simulink model "apf_system_H2"  (R2025a)
settings: Solver=FixedStepDiscrete  StartTime=0.0  StopTime=T_end  FixedStep=Tps  RelTol=1e-3
PostLoadFcn:
  | addpath(fileparts(get_param('apf_system_H2','FileName'))); if ~exist('P','var'), run(fullfile(fileparts(get_param('apf_system_H2','FileName')),'apf_params.m')); end; if ~exist('S','var'), S = sensor_params_H2; end
InitFcn:
  | addpath(fileparts(get_param('apf_system_H2','FileName'))); if ~exist('P','var'), run(fullfile(fileparts(get_param('apf_system_H2','FileName')),'apf_params.m')); end; if ~exist('S','var'), S = sensor_params_H2; end
values from neighbouring files (symbols this model uses):
  Cdc = 1000e-6    (= 0.001)    [apf_params.m]
  dtc = Td / (Ts / 2) / 2    [apf_params.m]    (also in vps_vectors_H3.m = 0.02)
  f = 50    [apf_params.m]    (also in frontend_sizing_H1.m = fieldnames(opt); sensor_adc_study_H1.m = fullfile(outdir, ['seed777_' s{1} '.csv']); sensor_adc_study_H2.m = fullfile(outdir, [scen{k, 1} '.mat']))
  Lac_load = 0.5e-3    (= 0.0005)    [apf_params.m]
  Ldc_load = 20e-3    (= 0.02)    [apf_params.m]
  Lf = 3e-3    (= 0.003)    [apf_params.m]
  Lgrid = 10e-6    (= 1e-05)    [apf_params.m]
  R_load1 = 33    [apf_params.m]
  R_step = R_load1 * R_load2 / (R_load1 - R_load2)    (= 66)    [apf_params.m]
  Rac_load = 0.01    [apf_params.m]
  Rf = 0.1    [apf_params.m]
  Rgrid = 1e-3    (= 0.001)    [apf_params.m]
  Rleak = 20e3    (= 20000)    [apf_params.m]
  S = struct('tau', [o.tauV o.tauV o.tauI o.tauI o.tauI o.tauI o.tauDC],      'delay', o.delay, 'skew', o.skew, 'conv', o.conv, 'noise', o.noise,      'seed', o.seed, 'adc', logical(o.adc))    [sensor_params_H2.m]    (also in thd_table_H3.m = round(2^15 * sin(2 * pi * m / 200)); vps_rtl_check_H3.m = load(fullfile(outdir, 'vps_runs.mat')))
  T_log = 10e-6    (= 1e-05)    [apf_params.m]
  t_run = 0.01    [apf_params.m]
  t_step = 0.7    [apf_params.m]
  Tps = 0.5e-6    (= 5e-07)    [apf_params.m]    (also in sensor_params_H2.m)
  Ts = P.Ts    [apf_params.m]    (also in sensor_params_H2.m = 0.0001)
  Vll_rms = Vm * sqrt(3) / sqrt(2)    [apf_params.m]
libraries: spsSeriesRLCBranchLib x5, spsThreePhaseVIMeasurementLib x3, spsUniversalBridgeLib x2, spsThreePhaseSeriesRLCBranchLib x2, spsThreePhaseBreakerLib x1, simulink x1, spsThreePhaseSourceLib x1, spsBreakerLib x1, spsVoltageMeasurementLib x1, spspowerguiLib x1
settings Model: Creator=HeKe  LastModifiedBy=HeKe

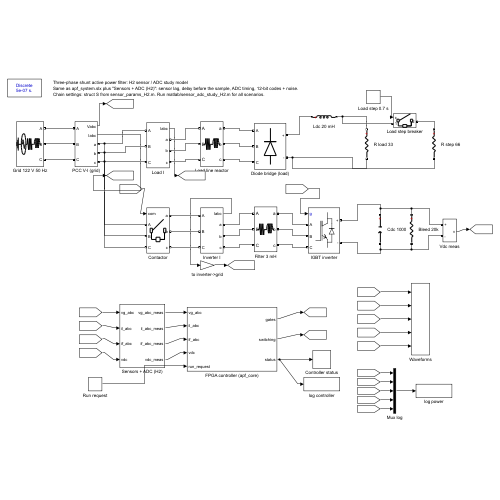
[thumbnail: Simulink's stored preview of the top-level diagram]
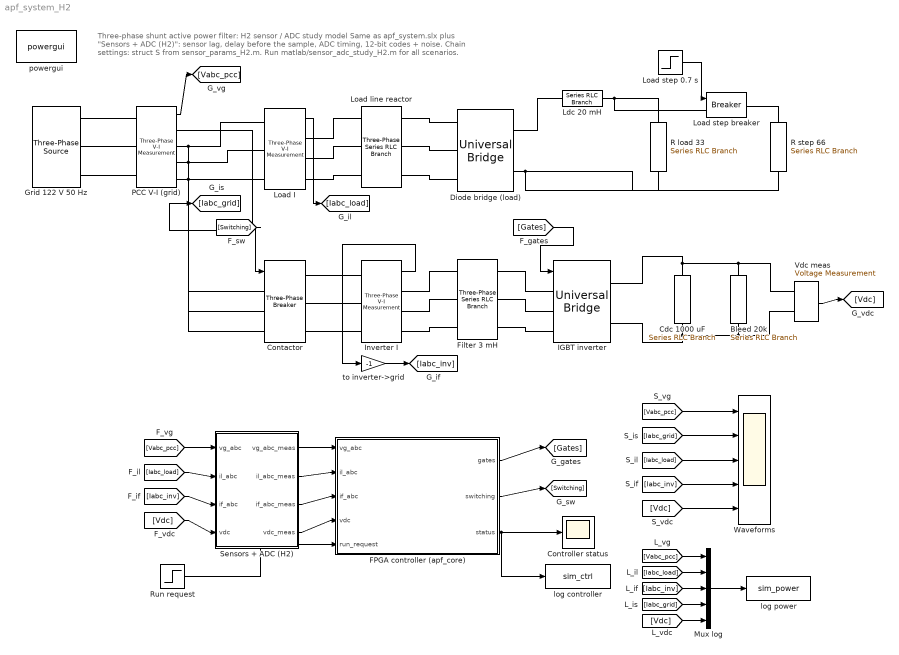
== system apf_system_H2 ==
  note: Three-phase shunt active power filter: H2 sensor / ADC study model
      | Same as apf_system.slx plus "Sensors + ADC (H2)": sensor lag, delay before the sample, ADC timing, 12-bit codes + noise.
      | Chain settings: struct S from sensor_params_H2.m. Run matlab/sensor_adc_study_H2.m for all scenarios.
  Bleed 20k : spsSeriesRLCBranchLib/Series RLC Branch  LConnTagsString=__new0  RConnTagsString=__new0  BranchType=R  Resistance=Rleak  Inductance=1e-3  SetiL0=off  InitialCurrent=0  Capacitance=1e-6  Setx0=off  InitialVoltage=0  Measurements=None
  Cdc 1000 uF : spsSeriesRLCBranchLib/Series RLC Branch  LConnTagsString=__new0  RConnTagsString=__new0  BranchType=C  Resistance=1  Inductance=1e-3  SetiL0=off  InitialCurrent=0  Capacitance=Cdc  Setx0=on  InitialVoltage=Vdc0  Measurements=None
  Contactor : spsThreePhaseBreakerLib/Three-Phase Breaker  InitialState=open  SwitchA=on  SwitchB=on  SwitchC=on  SwitchTimes="[1/60  5/60]"  External=on  BreakerResistance=1e-3  SnubberResistance=1e6  SnubberCapacitance=inf  Measurements=None
  Controller status : Scope
  Diode bridge (load) : spsUniversalBridgeLib/Universal Bridge  Arms=3  SnubberResistance=1e5  SnubberCapacitance=inf  Device=Diodes  Ron=Ron_sw  Lon=0  ForwardVoltages="[  0  0  ]"  ForwardVoltage=0  GTOparameters=[ 10e-6 , 20e-6 ]  IGBTparameters=[ 1e-6 , 2e-6 ]  Measurements=None  Measurements_2=None  converterType=Rectifier
  FPGA controller (apf_core) : Subsystem
  Filter 3 mH : spsThreePhaseSeriesRLCBranchLib/Three-Phase Series RLC Branch  LConnTagsString=A|B|C  RConnTagsString=A|B|C  BranchType=RL  Resistance=Rf  Inductance=Lf  Capacitance=1e-6  Measurements=None
  Grid 122 V 50 Hz : spsThreePhaseSourceLib/Three-Phase Source  InternalConnection=Yg  VoltagePhases=off  Voltage=Vll_rms  PhaseAngle=90  Voltage_phases=[25e3 25e3 25e3]/sqrt(3)  PhaseAngles_phases=[0 -120 +120]  Frequency=f  NonIdealSource=on  SpecifyImpedance=off  Resistance=Rgrid  Inductance=Lgrid  ShortCircuitLevel=100e6  BaseVoltage=25e3  XRratio=7  BusType=swing  Pref=10e3  Qref=0  Prefabc=[10e3, 10e3, 10e3]  Qrefabc=[0, 0, 0]  Qmin=-inf  Qmax=inf
  IGBT inverter : spsUniversalBridgeLib/Universal Bridge  Arms=3  SnubberResistance=1e5  SnubberCapacitance=inf  Device=IGBT / Diodes  Ron=Ron_sw  Lon=0  ForwardVoltages=[0 0]  ForwardVoltage=0  GTOparameters=[ 10e-6 , 20e-6 ]  IGBTparameters=[ 1e-6 , 2e-6 ]  Measurements=None  Measurements_2=None  converterType=Rectifier
  Inverter I : spsThreePhaseVIMeasurementLib/Three-Phase V-I Measurement  VoltageMeasurement=no  SetLabelV=off  LabelV=Vabc  Vpu=off  VpuLL=off  CurrentMeasurement=yes  SetLabelI=off  LabelI=Iabc  Ipu=off  Pbase=100e6  Vbase=500e3  OutputType=Complex  PhasorSimulation=off  PSBequivalent=0
  Ldc 20 mH : spsSeriesRLCBranchLib/Series RLC Branch  LConnTagsString=__new0  RConnTagsString=__new0  BranchType=L  Resistance=1  Inductance=Ldc_load  SetiL0=off  InitialCurrent=0  Capacitance=1e-6  Setx0=off  InitialVoltage=0  Measurements=None
  Load I : spsThreePhaseVIMeasurementLib/Three-Phase V-I Measurement  VoltageMeasurement=no  SetLabelV=off  LabelV=Vabc  Vpu=off  VpuLL=off  CurrentMeasurement=yes  SetLabelI=off  LabelI=Iabc  Ipu=off  Pbase=100e6  Vbase=500e3  OutputType=Complex  PhasorSimulation=off  PSBequivalent=0
  Load line reactor : spsThreePhaseSeriesRLCBranchLib/Three-Phase Series RLC Branch  LConnTagsString=A|B|C  RConnTagsString=A|B|C  BranchType=RL  Resistance=Rac_load  Inductance=Lac_load  Capacitance=1e-6  Measurements=None
  Load step 0.7 s : Step  Time=t_step  SampleTime=Ts
  Load step breaker : spsBreakerLib/Breaker  InitialState=0  SwitchingTimes="[1/60  5/60]"  External=on  BreakerResistance=1e-3  SnubberResistance=1e6  SnubberCapacitance=inf  Measurements=None  MoreParameters=on  NoBreakLoop=off
  Mux log : Mux  Inputs=[3 3 3 3 1]
  PCC V-I (grid) : spsThreePhaseVIMeasurementLib/Three-Phase V-I Measurement  VoltageMeasurement=phase-to-ground  SetLabelV=off  LabelV=Vabc  Vpu=off  VpuLL=off  CurrentMeasurement=yes  SetLabelI=off  LabelI=Iabc  Ipu=off  Pbase=100e6  Vbase=500e3  OutputType=Complex  PhasorSimulation=off  PSBequivalent=0
  R load 33 : spsSeriesRLCBranchLib/Series RLC Branch  LConnTagsString=__new0  RConnTagsString=__new0  BranchType=R  Resistance=R_load1  Inductance=1e-3  SetiL0=off  InitialCurrent=0  Capacitance=1e-6  Setx0=off  InitialVoltage=0  Measurements=None
  R step 66 : spsSeriesRLCBranchLib/Series RLC Branch  LConnTagsString=__new0  RConnTagsString=__new0  BranchType=R  Resistance=R_step  Inductance=1e-3  SetiL0=off  InitialCurrent=0  Capacitance=1e-6  Setx0=off  InitialVoltage=0  Measurements=None
  Run request : Step  Time=t_run  SampleTime=Ts
  Sensors + ADC (H2) : Subsystem
  Vdc meas : spsVoltageMeasurementLib/Voltage Measurement  PhasorSimulation=off  OutputType=Complex  PSBequivalent=0
  Waveforms : Scope  NumInputPorts=5
  log controller : ToWorkspace  VariableName=sim_ctrl  SaveFormat=Structure With Time  SampleTime=Ts
  log power : ToWorkspace  VariableName=sim_power  SaveFormat=Structure With Time  SampleTime=T_log
  powergui : spspowerguiLib/powergui  Priority=1  SimulationMode=Discrete  SampleTime=Tps  frequency=60  Iterations=50  frequencyindice=60  Pbase=100e6  ErrMax=1e-4  UnitsV=kV  UnitsW=MW  buscounter=0  FunctionMessages=off  echomessages=off  EnableUseOfTLC=off  CurrentSourceSwitches=off  DisableSnubberDevices=off  DisableRonSwitches=off  DisableVfSwitches=off  DisplayEquations=off  AutomaticDiscreteSolvers=off  SolverType=Tustin/Backward Euler (TBE)  Interpol=off  ExternalGateDelay=off  methode=off  Ts=100  x0status=blocks  SPID=on  SwTol=0  HookPort=off  NonlinearTolerance=1e-4  nMaxIteration=100  ContinueOnMaxIteration=off  RestoreLinks=warning  ResistiveCurrentMeasurement=off  Frange=[0:2:500]  Ylog=off  Xlog=on  ShowGrid=off  save=off  variable=ZData  structure=0  ZoomFFT=off  StartTime=0.0  cycles=1  DisplayStyle=1  fundamental=60  FreqAxis=off  MaxFrequency=1000  frequencyindicesteady=1  RmsSteady=1  display=off
  to inverter->grid : Gain  Gain=-1
  wires:
  Load step 0.7 s/1 -> Load step breaker/1
  PCC V-I (grid)/1 -> [Vabc_pcc]
  PCC V-I (grid)/2 -> [Iabc_grid]
  Load I/1 -> [Iabc_load]
  Inverter I/1 -> to inverter->grid/1
  to inverter->grid/1 -> [Iabc_inv]
  Vdc meas/1 -> [Vdc]
  [Gates] -> IGBT inverter/1
  [Switching] -> Contactor/1
  FPGA controller (apf_core)/1(gates) -> [Gates]
  FPGA controller (apf_core)/2(switching) -> [Switching]
  [Vabc_pcc] -> Waveforms/1
  [Iabc_grid] -> Waveforms/2
  [Iabc_load] -> Waveforms/3
  [Iabc_inv] -> Waveforms/4
  [Vdc] -> Waveforms/5
  [Vabc_pcc] -> Mux log/1
  [Iabc_load] -> Mux log/2
  [Iabc_inv] -> Mux log/3
  [Iabc_grid] -> Mux log/4
  [Vdc] -> Mux log/5
  Mux log/1 -> log power/1
  FPGA controller (apf_core)/3(status) -> Controller status/1, log controller/1
  Run request/1 -> FPGA controller (apf_core)/5(run_request)
  [Vabc_pcc] -> Sensors + ADC (H2)/1(vg_abc)
  Sensors + ADC (H2)/1(vg_abc_meas) -> FPGA controller (apf_core)/1(vg_abc)
  [Iabc_load] -> Sensors + ADC (H2)/2(il_abc)
  Sensors + ADC (H2)/2(il_abc_meas) -> FPGA controller (apf_core)/2(il_abc)
  [Iabc_inv] -> Sensors + ADC (H2)/3(if_abc)
  Sensors + ADC (H2)/3(if_abc_meas) -> FPGA controller (apf_core)/3(if_abc)
  [Vdc] -> Sensors + ADC (H2)/4(vdc)
  Sensors + ADC (H2)/4(vdc_meas) -> FPGA controller (apf_core)/4(vdc)
  connections:
  Grid 122 V 50 Hz/RConn1 -- PCC V-I (grid)/LConn1
  Load I/LConn1 -- PCC V-I (grid)/RConn1 -- Contactor/LConn1
  Load I/RConn1 -- Load line reactor/LConn1
  Load line reactor/RConn1 -- Diode bridge (load)/LConn1
  Contactor/RConn1 -- Inverter I/LConn1
  Inverter I/RConn1 -- Filter 3 mH/LConn1
  Filter 3 mH/RConn1 -- IGBT inverter/LConn1
  Grid 122 V 50 Hz/RConn2 -- PCC V-I (grid)/LConn2
  Load I/LConn2 -- PCC V-I (grid)/RConn2 -- Contactor/LConn2
  Load I/RConn2 -- Load line reactor/LConn2
  Load line reactor/RConn2 -- Diode bridge (load)/LConn2
  Contactor/RConn2 -- Inverter I/LConn2
  Inverter I/RConn2 -- Filter 3 mH/LConn2
  Filter 3 mH/RConn2 -- IGBT inverter/LConn2
  Grid 122 V 50 Hz/RConn3 -- PCC V-I (grid)/LConn3
  Load I/LConn3 -- PCC V-I (grid)/RConn3 -- Contactor/LConn3
  Load I/RConn3 -- Load line reactor/LConn3
  Load line reactor/RConn3 -- Diode bridge (load)/LConn3
  Contactor/RConn3 -- Inverter I/LConn3
  Inverter I/RConn3 -- Filter 3 mH/LConn3
  Filter 3 mH/RConn3 -- IGBT inverter/LConn3
  Diode bridge (load)/RConn1 -- Ldc 20 mH/LConn1
  R load 33/LConn1 -- Ldc 20 mH/RConn1 -- Load step breaker/LConn1
  Load step breaker/RConn1 -- R step 66/LConn1
  Diode bridge (load)/RConn2 -- R load 33/RConn1 -- R step 66/RConn1
  Cdc 1000 uF/LConn1 -- IGBT inverter/RConn1 -- Bleed 20k/LConn1 -- Vdc meas/LConn1
  Cdc 1000 uF/RConn1 -- IGBT inverter/RConn2 -- Bleed 20k/RConn1 -- Vdc meas/LConn2

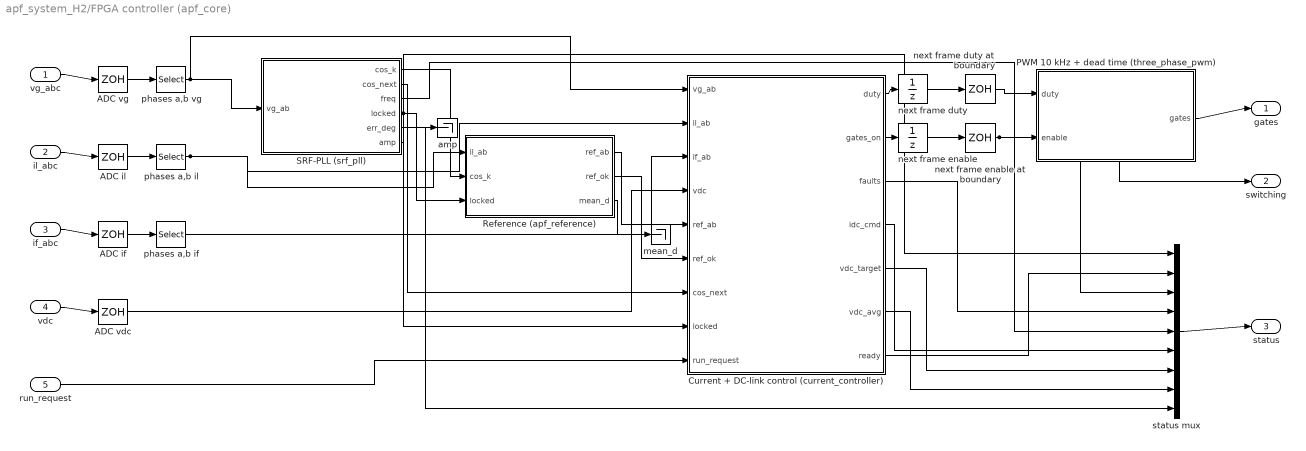
== system apf_system_H2/FPGA controller (apf_core) ==
  vg_abc : Inport
  il_abc : Inport  Port=2
  if_abc : Inport  Port=3
  vdc : Inport  Port=4
  run_request : Inport  Port=5
  ADC if : ZeroOrderHold  SampleTime=[Ts S.conv]
  ADC il : ZeroOrderHold  SampleTime=[Ts S.conv]
  ADC vdc : ZeroOrderHold  SampleTime=[Ts S.conv]
  ADC vg : ZeroOrderHold  SampleTime=[Ts S.conv]
  Current + DC-link control (current_controller) : MATLAB Function  TreatAsAtomicUnit=on  SystemSampleTime=[Ts S.conv]
  PWM 10 kHz + dead time (three_phase_pwm) : Subsystem
  Reference (apf_reference) : MATLAB Function  TreatAsAtomicUnit=on  SystemSampleTime=[Ts S.conv]
  SRF-PLL (srf_pll) : MATLAB Function  TreatAsAtomicUnit=on  SystemSampleTime=[Ts S.conv]
  amp : Terminator
  mean_d : Terminator
  next frame duty : UnitDelay  SampleTime=Tps  HasFrameUpgradeWarning=on
  next frame duty at boundary : ZeroOrderHold  SampleTime=Ts
  next frame enable : UnitDelay  SampleTime=Tps  HasFrameUpgradeWarning=on
  next frame enable at boundary : ZeroOrderHold  SampleTime=Ts
  phases a,b if : Selector  InputPortWidth=3  IndexOptions=Index vector (dialog)  Indices=[1 2]  OutputSizes=1
  phases a,b il : Selector  InputPortWidth=3  IndexOptions=Index vector (dialog)  Indices=[1 2]  OutputSizes=1
  phases a,b vg : Selector  InputPortWidth=3  IndexOptions=Index vector (dialog)  Indices=[1 2]  OutputSizes=1
  status mux : Mux  Inputs=[1 1 1 4 1 1 1 1 1]
  gates : Outport
  switching : Outport  Port=2
  status : Outport  Port=3
  wires:
  vg_abc/1 -> ADC vg/1
  ADC vg/1 -> phases a,b vg/1
  il_abc/1 -> ADC il/1
  ADC il/1 -> phases a,b il/1
  if_abc/1 -> ADC if/1
  ADC if/1 -> phases a,b if/1
  vdc/1 -> ADC vdc/1
  phases a,b vg/1 -> SRF-PLL (srf_pll)/1(vg_ab), Current + DC-link control (current_controller)/1(vg_ab)
  phases a,b il/1 -> Reference (apf_reference)/1(il_ab), Current + DC-link control (current_controller)/2(il_ab)
  SRF-PLL (srf_pll)/1(cos_k) -> Reference (apf_reference)/2(cos_k)
  SRF-PLL (srf_pll)/4(locked) -> Reference (apf_reference)/3(locked), Current + DC-link control (current_controller)/8(locked), status mux/1
  phases a,b if/1 -> Current + DC-link control (current_controller)/3(if_ab)
  ADC vdc/1 -> Current + DC-link control (current_controller)/4(vdc)
  Reference (apf_reference)/1(ref_ab) -> Current + DC-link control (current_controller)/5(ref_ab)
  Reference (apf_reference)/2(ref_ok) -> Current + DC-link control (current_controller)/6(ref_ok)
  SRF-PLL (srf_pll)/2(cos_next) -> Current + DC-link control (current_controller)/7(cos_next)
  run_request/1 -> Current + DC-link control (current_controller)/9(run_request)
  Current + DC-link control (current_controller)/1(duty) -> next frame duty/1
  Current + DC-link control (current_controller)/2(gates_on) -> next frame enable/1
  PWM 10 kHz + dead time (three_phase_pwm)/1(gates) -> gates/1
  Current + DC-link control (current_controller)/7(ready) -> status mux/2
  Current + DC-link control (current_controller)/3(faults) -> status mux/4
  SRF-PLL (srf_pll)/3(freq) -> status mux/5
  Current + DC-link control (current_controller)/4(idc_cmd) -> status mux/6
  Current + DC-link control (current_controller)/5(vdc_target) -> status mux/7
  Current + DC-link control (current_controller)/6(vdc_avg) -> status mux/8
  SRF-PLL (srf_pll)/5(err_deg) -> status mux/9
  status mux/1 -> status/1
  SRF-PLL (srf_pll)/6(amp) -> amp/1
  Reference (apf_reference)/3(mean_d) -> mean_d/1
  next frame duty/1 -> next frame duty at boundary/1
  next frame duty at boundary/1 -> PWM 10 kHz + dead time (three_phase_pwm)/1(duty)
  next frame enable/1 -> next frame enable at boundary/1
  next frame enable at boundary/1 -> PWM 10 kHz + dead time (three_phase_pwm)/2(enable), switching/1, status mux/3

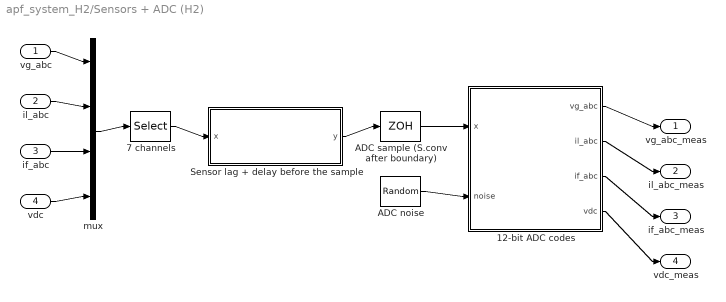
== system apf_system_H2/Sensors + ADC (H2) ==
  vg_abc : Inport
  il_abc : Inport  Port=2
  if_abc : Inport  Port=3
  vdc : Inport  Port=4
  12-bit ADC codes : MATLAB Function  TreatAsAtomicUnit=on
  7 channels : Selector  InputPortWidth=10  IndexOptions=Index vector (dialog)  Indices=[1 2 4 5 7 8 10]  OutputSizes=1
  ADC noise : RandomNumber  Mean=zeros(7,1)  Seed=S.seed + (0:6)'  SampleTime=[Ts S.conv]
  ADC sample (S.conv after boundary) : ZeroOrderHold  SampleTime=[Ts S.conv]
  Sensor lag + delay before the sample : MATLAB Function  TreatAsAtomicUnit=on  SystemSampleTime=Tps
  mux : Mux  Inputs=[3 3 3 1]
  vg_abc_meas : Outport
  il_abc_meas : Outport  Port=2
  if_abc_meas : Outport  Port=3
  vdc_meas : Outport  Port=4
  wires:
  vg_abc/1 -> mux/1
  il_abc/1 -> mux/2
  if_abc/1 -> mux/3
  vdc/1 -> mux/4
  mux/1 -> 7 channels/1
  7 channels/1 -> Sensor lag + delay before the sample/1(x)
  Sensor lag + delay before the sample/1(y) -> ADC sample (S.conv after boundary)/1
  ADC sample (S.conv after boundary)/1 -> 12-bit ADC codes/1(x)
  ADC noise/1 -> 12-bit ADC codes/2(noise)
  12-bit ADC codes/1(vg_abc) -> vg_abc_meas/1
  12-bit ADC codes/2(il_abc) -> il_abc_meas/1
  12-bit ADC codes/3(if_abc) -> if_abc_meas/1
  12-bit ADC codes/4(vdc) -> vdc_meas/1

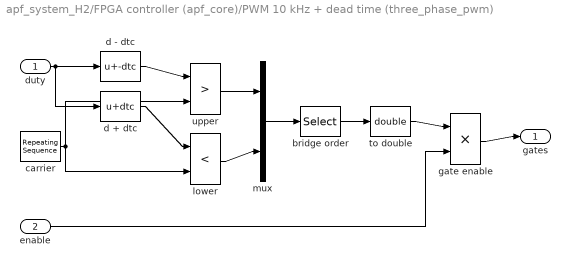
== system apf_system_H2/FPGA controller (apf_core)/PWM 10 kHz + dead time (three_phase_pwm) ==
  duty : Inport
  enable : Inport  Port=2
  bridge order : Selector  InputPortWidth=6  IndexOptions=Index vector (dialog)  Indices=[1 4 2 5 3 6]  OutputSizes=1
  carrier : simulink/Sources/Repeating Sequence  rep_seq_t=[0 Ts/2 Ts]  rep_seq_y=[0 1 0]
  d + dtc : Bias  Bias=dtc  SaturateOnIntegerOverflow=off
  d - dtc : Bias  Bias=-dtc  SaturateOnIntegerOverflow=off
  gate enable : Product
  lower : RelationalOperator  Operator=<  OutDataTypeStr=boolean  RndMeth=Simplest  InputSameDT=off
  mux : Mux  Inputs=2
  to double : DataTypeConversion  OutDataTypeStr=double  SaturateOnIntegerOverflow=off  RndMeth=Floor
  upper : RelationalOperator  Operator=>  OutDataTypeStr=boolean  RndMeth=Simplest  InputSameDT=off
  gates : Outport
  wires:
  duty/1 -> d - dtc/1, d + dtc/1
  d - dtc/1 -> upper/1
  carrier/1 -> upper/2, lower/2
  d + dtc/1 -> lower/1
  upper/1 -> mux/1
  lower/1 -> mux/2
  mux/1 -> bridge order/1
  bridge order/1 -> to double/1
  to double/1 -> gate enable/1
  enable/1 -> gate enable/2
  gate enable/1 -> gates/1

== matlab function apf_system_H2/FPGA controller (apf_core)/Reference (apf_reference) ==
  data: il_ab input; ref_ab output; cos_k input; locked input; ref_ok output; mean_d output; P parameter
function [ref_ab, ref_ok, mean_d] = apf_reference_block(il_ab, cos_k, locked, P)
% Compensation reference, floating-point equivalent of rtl/apf_reference.sv.
%   d      = 2/3 * sum(i_load_p * cos_p)       (active load current, this sample)
%   mean_d = average of d over one grid cycle   (N samples)
%   ref_p  = i_load_p - mean_d * cos_p          (harmonics + reactive current)
% The history is discarded whenever the PLL is not locked.
persistent hist idx cnt total
NMAX = 400;                       % buffer size; P.N must not exceed it
if isempty(hist)
    hist = zeros(1, NMAX); idx = 1; cnt = 0; total = 0;
end
ref_ab = [0, 0];
ref_ok = 0;
mean_d = 0;
if locked < 0.5
    hist(:) = 0; idx = 1; cnt = 0; total = 0;
    return;
end
N = P.N;
il = [il_ab(1), il_ab(2), -(il_ab(1) + il_ab(2))];
d = 2/3 * sum(il .* cos_k);

% Rolling sum over the last N samples.
if cnt == N
    total = total - hist(idx);
end
total = total + d;
hist(idx) = d;
idx = idx + 1;
if idx > N, idx = 1; end
cnt = min(cnt + 1, N);

if cnt == N
    mean_d = total / N;
    ref_ab = il(1:2) - mean_d * cos_k(1:2);
    ref_ok = 1;
end

== matlab function apf_system_H2/FPGA controller (apf_core)/SRF-PLL (srf_pll) ==
  data: vg_ab input; cos_k output; cos_next output; freq output; locked output; err_deg output; amp output; P parameter
function [cos_k, cos_next, freq, locked, err_deg, amp] = srf_pll_block(vg_ab, P)
% Three-phase SRF-PLL, floating-point equivalent of rtl/srf_pll.sv
% (bit-exact integer model: model/pll_model.py). Runs once per control frame.
%   cos_k    cosines of the angle predicted for this sample (used by the reference)
%   cos_next cosines for the next sample (used by the current controller)
persistent theta integ is_locked lock_cnt unlock_cnt
if isempty(theta)
    theta = 0; integ = 0; is_locked = false; lock_cnt = 0; unlock_cnt = 0;
end
sh = [0, -2*pi/3, 2*pi/3];
vabc = [vg_ab(1), vg_ab(2), -(vg_ab(1) + vg_ab(2))];

% 1. Park transform with the predicted angle.
c = cos(theta + sh);
s = sin(theta + sh);
vd = 2/3 * sum(vabc .* c);
vq = -2/3 * sum(vabc .* s);

% 2. Normalise q by the magnitude: error = sin(phase error).
amp = sqrt(vd^2 + vq^2);
low_amp = amp < P.pll_vmin;
e = 0;
if ~low_amp
    e = vq / amp;
end

% 3. PI loop with frequency clamp and anti-windup.
wn = 2*pi*P.pll_bw;
kp = 2*P.pll_zeta*wn;
ki = wn^2;
imax = 2*pi*(P.pll_fmax - P.f);
integ = min(max(integ + ki*e*P.Ts, -imax), imax);
w = min(max(2*pi*P.f + kp*e + integ, 2*pi*P.pll_fmin), 2*pi*P.pll_fmax);

% 4. Advance the angle for the next sample.
theta = mod(theta + w*P.Ts, 2*pi);

% 5. Lock detection.
good = ~low_amp && abs(e) <= sin(P.lock_deg*pi/180);
bad  = low_amp || abs(e) > sin(P.unlock_deg*pi/180);
if ~is_locked
    if good, lock_cnt = lock_cnt + 1; else, lock_cnt = 0; end
    if lock_cnt >= P.lock_n
        is_locked = true; unlock_cnt = 0;
    end
else
    if bad, unlock_cnt = unlock_cnt + 1; else, unlock_cnt = 0; end
    if unlock_cnt >= P.unlock_n
        is_locked = false; lock_cnt = 0;
    end
end

cos_k = c;
cos_next = cos(theta + sh);
freq = w / (2*pi);
locked = double(is_locked);
err_deg = asin(e) * 180/pi;

== matlab function apf_system_H2/FPGA controller (apf_core)/Current + DC-link control (current_controller) ==
  data: vg_ab input; duty output; il_ab input; if_ab input; vdc input; ref_ab input; ref_ok input; cos_next input; locked input; run_request input; gates_on output; faults output; idc_cmd output; vdc_target output; vdc_avg output; ready output; P parameter
function [duty, gates_on, faults, idc_cmd, vdc_target, vdc_avg, ready] = apf_control_block( ...
    vg_ab, il_ab, if_ab, vdc, ref_ab, ref_ok, cos_next, locked, run_request, P)
% Predictive (deadbeat) current control, DC-link loop, protection and start-up
% sequencing: floating-point equivalent of rtl/current_controller.sv and the
% sequencing in rtl/apf_core.sv. Runs once per control frame k.
%   duty     upper-switch on fraction per phase, applied over [k+1, k+2]
%   gates_on inverter switching (and contactor) enable for the same interval
%   faults   latched [measurement, over_current, over_voltage, pll_lost]
persistent raw vg_prev hist wr fill vdc_sum vdc_cnt avg vdc_avg_ok integ idc vtgt fresh run_ctrl fault_q
NMAX = 400;
if isempty(raw)
    raw = [0.5, 0.5, 0.5]; vg_prev = [0, 0];
    hist = zeros(2, NMAX); wr = 1; fill = 0;
    vdc_sum = 0; vdc_cnt = 0; avg = 0; vdc_avg_ok = false;
    integ = 0; idc = 0; vtgt = 0;
    fresh = true; run_ctrl = false; fault_q = false(1, 4);
end
N = P.N; Ts = P.Ts; L = P.Lf;
vg3 = [vg_ab(1), vg_ab(2), -(vg_ab(1) + vg_ab(2))];
il3 = [il_ab(1), il_ab(2), -(il_ab(1) + il_ab(2))];
if3 = [if_ab(1), if_ab(2), -(if_ab(1) + if_ab(2))];

% ---- protection and sequencing (apf_core) ----
fault_now = [any(abs(vg3(1:2)) > P.v_range) || any(abs(il3(1:2)) > P.i_range) || ...
                 any(abs(if3(1:2)) > P.i_range), ...
             any(abs(if3) > P.i_trip), ...
             vdc > P.vdc_trip, ...
             run_ctrl && locked < 0.5];
% The controller sees the run decision registered in an earlier frame.
run_q = run_ctrl && fill == N && ref_ok > 0.5 && vdc_avg_ok;
if run_request < 0.5
    run_ctrl = false;                     % dropping the request clears faults
    fault_q(:) = false;
elseif any(fault_q) || any(fault_now)
    fault_q = fault_q | fault_now;        % latch, stop switching
    run_ctrl = false;
elseif ~run_ctrl && fill == N && vdc_avg_ok && locked > 0.5
    run_ctrl = true;
end
run_q = run_q && run_ctrl;

% ---- 1. predict the filter current at k+1 ----
dv = vg_ab(:)' - vg_prev;
u_prev = vdc * (raw(1:2) - mean(raw));    % differential voltage applied over [k, k+1]
e1 = u_prev - vg_ab(:)' - dv/2;
if fresh                                   % inverter was not switching over [k, k+1]
    i_pred = if_ab(:)';
else
    i_pred = if_ab(:)' + Ts/L * e1;
end
i_pred3 = [i_pred, -(i_pred(1) + i_pred(2))];

% ---- 2. reference for k+2: one grid cycle earlier, minus the DC-link term ----
rd = wr + P.pred_lead;
if rd > N, rd = rd - N; end
rp = hist(:, rd)' - idc * cos_next(1:2);

% ---- 3. deadbeat voltage with grid feed-forward ----
u = vg_ab(:)' + 1.5*dv + P.G * L/Ts * (rp - i_pred);
u3 = [u, -(u(1) + u(2))];

% ---- 4. min/max common-mode injection, divide by Vdc, dead-time compensation ----
off = -(max(u3) + min(u3)) / 2;
vdc_div = max(vdc, P.vdc_min_div);
raw_n = min(max(0.5 + (u3 + off) / vdc_div, 0), 1);
vg_prev = vg_ab(:)';
if run_q
    raw = raw_n;
    duty = min(max(raw_n + P.Td/Ts * (2*(i_pred3 > 0) - 1), 0), 1);
    fresh = false;
else
    raw = [0.5, 0.5, 0.5];
    duty = [0.5, 0.5, 0.5];
    fresh = true;
end
gates_on = double(run_q);

% ---- store this frame's reference; drop the history if it is broken ----
if ref_ok > 0.5
    hist(:, wr) = ref_ab(:);
    wr = wr + 1;
    if wr > N, wr = 1; end
    fill = min(fill + 1, N);
else
    wr = 1; fill = 0;
end

% ---- DC-link PI, once per grid cycle on the cycle average ----
vdc_sum = vdc_sum + vdc;
vdc_cnt = vdc_cnt + 1;
if vdc_cnt == N
    avg = vdc_sum / N;
    vdc_sum = 0; vdc_cnt = 0; vdc_avg_ok = true;
    if ~run_q
        vtgt = avg; integ = 0; idc = 0;
    else
        vtgt = min(vtgt + P.vdc_ramp * N * Ts, P.vdc_ref);
        err = vtgt - avg;
        integ = min(max(integ + P.ki_dc * err * N * Ts, -P.idc_max), P.idc_max);
        idc = min(max(P.kp_dc * err + integ, -P.idc_max), P.idc_max);
    end
end

faults = double(fault_q);
idc_cmd = idc;
vdc_target = vtgt;
vdc_avg = avg;
ready = double(fill == N && vdc_avg_ok && locked > 0.5);

== matlab function apf_system_H2/Sensors + ADC (H2)/Sensor lag + delay before the sample ==
  data: x input; y output; S parameter; Tps parameter
function y = sensor_chain_block_H2(x, S, Tps)
% H2: sensors and the delay in front of the ADC, run at the power-stage step Tps.
%   x, y   [vg_a vg_b il_a il_b if_a if_b vdc]  (V, A, V); y is what the ADC samples
% Per channel:
%   - first-order sensor lag, time constant S.tau (0 = ideal sensor)
%   - pure delay S.delay before the sample (ADC anti-alias filter group delay,
%     delta-sigma decimation filter, ...)
%   - plus S.conv - ch*S.skew: the ADC block samples at S.conv after the carrier
%     boundary (when the codes reach the FPGA), so this extra delay makes channel ch
%     show its value at boundary + ch*S.skew (multiplexed ADC) or at the boundary
%     itself (simultaneous ADC, skew 0), as in sim/tb_apf_system_H1.sv.
persistent lag buf wr
NBUF = 4096;                            % 2.048 ms at Tps = 0.5 us
if isempty(lag)
    lag = x(:);                         % start settled at the first plant values
    buf = repmat(x(:), 1, NBUF);
    wr = 1;
end
a = 1 - exp(-Tps ./ S.tau(:));          % tau = 0 gives a = 1 (no lag)
lag = lag + a .* (x(:) - lag);
buf(:, wr) = lag;
y = zeros(7, 1);
for ch = 1:7
    n = round((S.delay + S.conv - (ch - 1) * S.skew) / Tps);
    rd = wr - n;
    if rd < 1, rd = rd + NBUF; end
    y(ch) = buf(ch, rd);
end
wr = wr + 1;
if wr > NBUF, wr = 1; end

== matlab function apf_system_H2/Sensors + ADC (H2)/12-bit ADC codes ==
  data: x input; vg_abc output; noise input; il_abc output; if_abc output; vdc output; S parameter
function [vg_abc, il_abc, if_abc, vdc] = adc_quantizer_block_H2(x, noise, S)
% H2: 12-bit ADC codes exactly as rtl/apf_core.sv receives them, converted back
% to volts and amperes for the floating-point controller.
%   grid voltage 16 counts/V and currents 100 counts/A, zero at code 2048;
%   DC link 10 counts/V, zero at code 0; S.noise counts rms of white noise.
% Phase c is -(a + b), as in apf_core (only phases a and b are measured).
gain = [16 16 100 100 100 100 10]';
offset = [2048 2048 2048 2048 2048 2048 0]';
if S.adc
    c = offset + gain .* x(:) + S.noise * noise(:);
    c = floor(min(max(c, 0), 4095) + 0.5);
    v = (c - offset) ./ gain;
else
    v = x(:);                           % ideal ADC: no quantization or noise
end
vg_abc = [v(1); v(2); -(v(1) + v(2))];
il_abc = [v(3); v(4); -(v(3) + v(4))];
if_abc = [v(5); v(6); -(v(5) + v(6))];
vdc = v(7);
